simulink model "simulink_flightgear_control_trim_wind_5"  (R2023a)
settings: Solver=VariableStepAuto  StartTime=0  StopTime=inf  FixedStep=0.1  RelTol=1e-3
values from neighbouring files (symbols this model uses):
  model = 'simulink_flightgear_control_trim_wind_5'    [traimcode.m]
  ms2kts = 1.943844492609    (= 1.94384449261)    [Boeing747model.m]    (also in engine.m)
undefined symbols (not defined in the file or in its folder): Earth, F, Light, m, MIL, Model, Newton, Raphson, Receive, s, Send, Unit, WGS84, Wind
libraries: simulink_extras x7, aerolibconvert2 x5, simulink x4, aerolibfltsims x3, shared6dof x1, aerolibasang x1, aerolibtransform2 x1, aerolibatmos2 x1, aerolibobsolete x1, aerolibwind2 x1
(part 2 of 2)

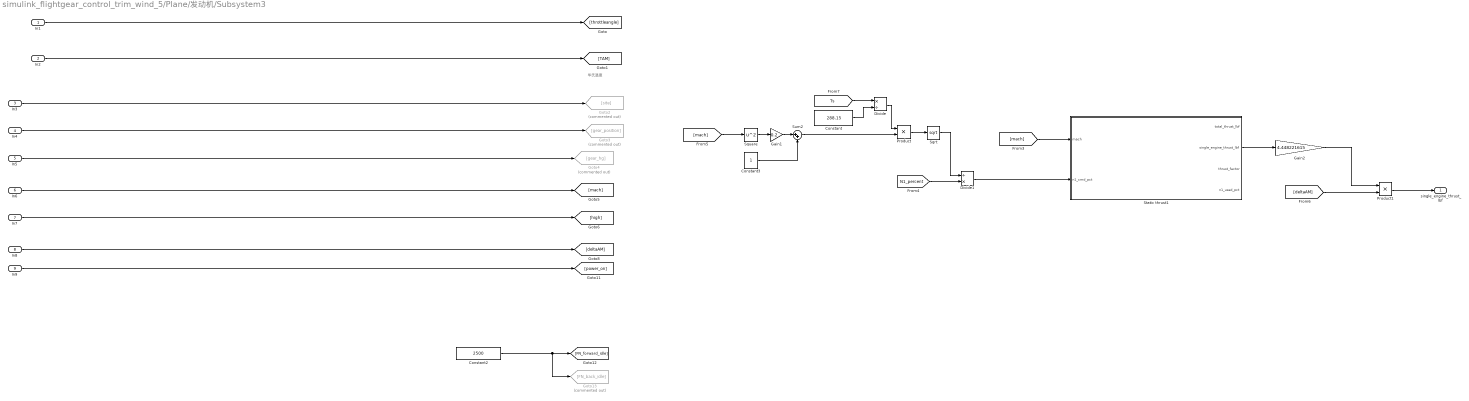
== system simulink_flightgear_control_trim_wind_5/Plane/发动机/Subsystem3 ==
  note: 华氏温度
  In1 : Inport
  In2 : Inport  Port=2
  In3 : Inport  Port=3
  In4 : Inport  Port=4
  In5 : Inport  Port=5
  In6 : Inport  Port=6
  In7 : Inport  Port=7
  In8 : Inport  Port=8
  In9 : Inport  Port=9
  Constant : Constant  Value=288.15
  Constant2 : Constant  Value=2500
  Constant3 : Constant
  Divide : Product  Inputs=*/
  Divide1 : Product  Inputs=/*
  Gain1 : Gain  Gain=0.2
  Gain2 : Gain  Gain=4.448221615
  Goto13 : Goto  Commented=on  GotoTag=FN_back_idle
  Goto2 : Goto  Commented=on  GotoTag=site
  Goto3 : Goto  Commented=on  GotoTag=gear_position
  Goto4 : Goto  Commented=on  GotoTag=gear_hg
  Product : Product
  Product1 : Product
  Sqrt : Sqrt
  Square : Math  Operator=square
  Static thrust1 : MATLAB Function  TreatAsAtomicUnit=on
  Sum2 : Sum  Inputs=|++
  single_engine_thrust_lbf : Outport
  wires:
  In2/1 -> [TAM]
  In1/1 -> [throttleangle]
  In5/1 -> Goto4/1
  In3/1 -> Goto2/1
  In4/1 -> Goto3/1
  In6/1 -> [mach]
  In8/1 -> [deltaAM]
  In7/1 -> [high]
  In9/1 -> [power_on]
  Constant2/1 -> [FN_forward_idle], Goto13/1
  Product1/1 -> single_engine_thrust_lbf/1
  [N1_percent] -> Divide1/2
  Divide1/1 -> Static thrust1/2(n1_cmd_pct)
  Divide/1 -> Product/1
  [mach] -> Square/1
  [Ts] -> Divide/1
  Constant3/1 -> Sum2/2
  [mach] -> Static thrust1/1(mach)
  Constant/1 -> Divide/2
  Gain1/1 -> Sum2/1
  Sum2/1 -> Product/2
  Square/1 -> Gain1/1
  Sqrt/1 -> Divide1/1
  Product/1 -> Sqrt/1
  [deltaAM] -> Product1/2
  Static thrust1/2(single_engine_thrust_lbf) -> Gain2/1
  Gain2/1 -> Product1/1

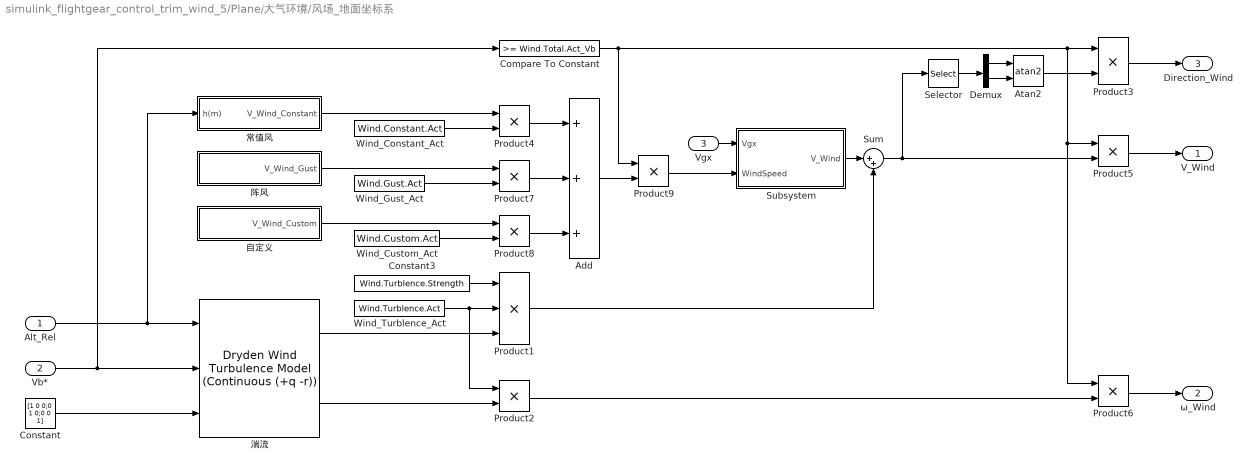
== system simulink_flightgear_control_trim_wind_5/Plane/大气环境/风场_地面坐标系 ==
  Alt_Rel : Inport
  Vb* : Inport  Port=2
  Vgx : Inport  Port=3
  Add : Sum  Inputs=+++
  Atan2 : Trigonometry  Operator=atan2
  Compare To Constant : simulink/Logic and Bit Operations/Compare To Constant  relop=>=  const=Wind.Total.Act_Vb  OutDataTypeStr=uint8
  Constant : Constant  Value=[1 0 0;0 1 0;0 0 1]
  Constant3 : Constant  Value=Wind.Turblence.Strength
  Demux : Demux  Outputs=2
  Product1 : Product  Inputs=3
  Product{2..9} (8 alike) : Product
  Selector : Selector  InputPortWidth=3  IndexOptions=Index vector (dialog)  Indices=[2 1]  OutputSizes=1
  Subsystem : Subsystem
  Sum : Sum  Inputs=|++
  Wind_Constant_Act : Constant  Value=Wind.Constant.Act
  Wind_Custom_Act : Constant  Value=Wind.Custom.Act
  Wind_Gust_Act : Constant  Value=Wind.Gust.Act
  Wind_Turblence_Act : Constant  Value=Wind.Turblence.Act
  常值风 : Subsystem
  湍流 : aerolibwind2/Dryden Wind Turbulence Model  (Continuous (+q -r))  units=Metric (MKS)  spec=MIL-F-8785C  model=Continuous Dryden (+q +r)  W20=Wind.Constant.Vxy_Ground  Wdeg=Wind.Constant.Direction  TurbProb=10^-2 - Light  L_high=533.4  Wingspan=Model.b  ts=Wind.Turblence.SampleTime  Seed=[fix(rand(1,1)*25000), fix(rand(1,1)*25000+1), fix(rand(1,1)*25000+2), fix(rand(1,1)*25000+3)]  T_on=on
  自定义 : Subsystem
  阵风 : Subsystem
  V_Wind : Outport  VectorParamsAs1DForOutWhenUnconnected=off
  ω_Wind : Outport  Port=2  VectorParamsAs1DForOutWhenUnconnected=off
  Direction_Wind : Outport  Port=3  VectorParamsAs1DForOutWhenUnconnected=off
  wires:
  Wind_Custom_Act/1 -> Product8/2
  Product8/1 -> Add/3
  自定义/1(V_Wind_Custom) -> Product8/1
  Wind_Turblence_Act/1 -> Product2/1, Product1/2
  Wind_Gust_Act/1 -> Product7/2
  Wind_Constant_Act/1 -> Product4/2
  Demux/1 -> Atan2/1
  Demux/2 -> Atan2/2
  Selector/1 -> Demux/1
  Compare To Constant/1 -> Product9/1, Product6/1, Product5/1, Product3/1
  Atan2/1 -> Product3/2
  Subsystem/1(V_Wind) -> Sum/1
  Sum/1 -> Product5/2, Selector/1
  Product7/1 -> Add/2
  阵风/1(V_Wind_Gust) -> Product7/1
  Product4/1 -> Add/1
  Product1/1 -> Sum/2
  Product3/1 -> Direction_Wind/1
  Product2/1 -> Product6/2
  Constant3/1 -> Product1/1
  Product6/1 -> ω_Wind/1
  Product5/1 -> V_Wind/1
  Constant/1 -> 湍流/3
  常值风/1(V_Wind_Constant) -> Product4/1
  Vb*/1 -> Compare To Constant/1, 湍流/2
  湍流/2 -> Product2/2
  湍流/1 -> Product1/3
  Alt_Rel/1 -> 常值风/1(h(m)), 湍流/1
  Vgx/1 -> Subsystem/1(Vgx)
  Product9/1 -> Subsystem/2(WindSpeed)
  Add/1 -> Product9/2

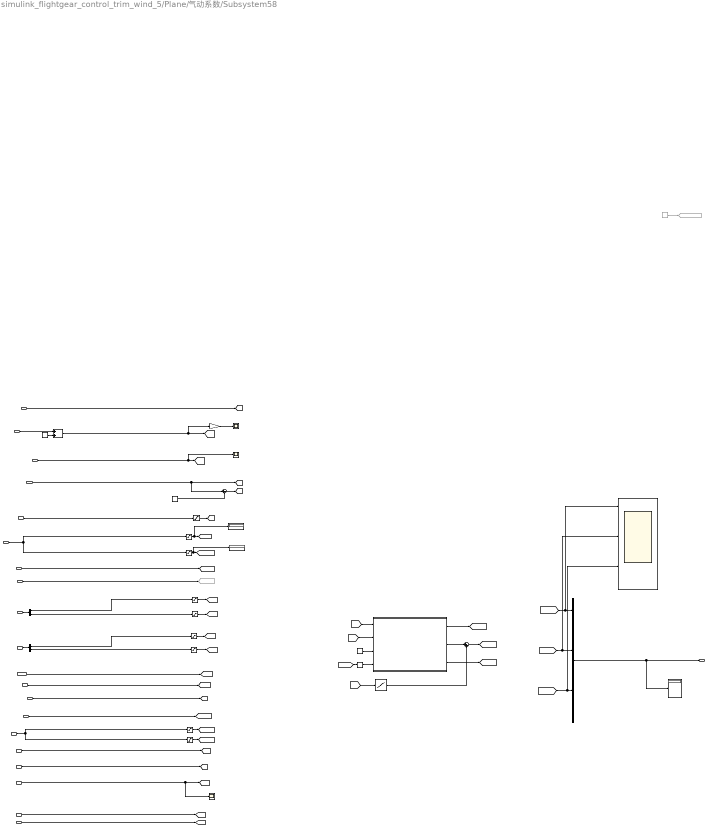
== system simulink_flightgear_control_trim_wind_5/Plane/气动系数/Subsystem58 ==
  note: degree
  note: 输入单位:
      | 角度：弧度
      | 角速度：rad/s
      | 速度:mach
      | 舵面：rad
      | 襟翼：0-1
      | 高度：米
      | 重心：百分比
  note: 内侧升降舵偏转角度
  note: 平尾配平角度
  note: 迎角RAD+安装角
      | 安装角
  note: 外侧升降舵偏转角度
  note: 起落架时间控制系统
  In1 : Inport
  In2 : Inport  Port=2
  In3 : Inport  Port=3
  In4 : Inport  Port=4
  In5 : Inport  Port=5
  In6 : Inport  Port=6
  trim : Inport  Port=7
  In8 : Inport  Port=8
  aere_o : Inport  Port=9
  In10 : Inport  Port=10
  In11 : Inport  Port=11
  In12 : Inport  Port=12
  In13 : Inport  Port=13
  In14 : Inport  Port=14
  In15 : Inport  Port=15
  In16 : Inport  Port=16
  In17 : Inport  Port=17
  In18 : Inport  Port=18
  V_E : Inport  Port=19
  In20 : Inport  Port=20
  2-D Lookup Table : Lookup_n-D  NumberOfTableDimensions=1  BreakpointsForDimension1="[0.0 0.2 0.3 0.4 0.5 0.6 0.7  0.8 0.9 1 1.1 1.2 1.3 3]"  BreakpointsForDimension2=[1:3]  Table="[0   0   0   0   0   0   0.002 0.008 0.02 0.045 0.08 0.045 0.03 0.03]"  InternalRulePriority=Speed  RndMeth=Simplest
  Bus Creator : BusCreator  Inputs=6
  Constant : Constant  Value=0.03490658504
  Constant11 : Constant  Value=0
  Constant4 : Constant  Value=4.58
  Constant5 : Constant  Commented=on  Value=0
  Degrees to Radians : simulink_extras/Transformations/Degrees to Radians
  Demux : Demux  Outputs=2
  Demux1 : Demux  Outputs=2
  Display : Display
  Display1 : Display
  Display2 : Display
  Gain1 : Gain  Gain=57.3
  Goto19 : Goto  Commented=on  GotoTag=gear_position
  Goto35 : Goto  Commented=on  GotoTag=K
  Saturation1 : Saturate  UpperLimit=0.26  LowerLimit=-0.436
  Saturation10 : Saturate  UpperLimit=0.26  LowerLimit=-0.436
  Saturation12 : Saturate  UpperLimit=33  LowerLimit=14
  Saturation14 : Saturate  UpperLimit=0.436  LowerLimit=-0.436
  Saturation16 : Saturate  UpperLimit=0.436  LowerLimit=-0.436
  Saturation3 : Saturate  UpperLimit=0.349  LowerLimit=-0.349
  Saturation4 : Saturate  UpperLimit=0.349  LowerLimit=-0.349
  Saturation8 : Saturate  UpperLimit=0.4  LowerLimit=-0.296
  Saturation9 : Saturate  UpperLimit=0.4  LowerLimit=-0.296
  Scope10 : Scope  NumInputPorts=6
  Scope11 : Scope
  Scope12 : Scope
  Scope16 : Scope
  Static longitudinal aero : MATLAB Function  TreatAsAtomicUnit=on
  Sum : Sum  Inputs=|++
  Sum13 : Sum  Inputs=|+-
  Sum5 : Sum
  Coefficients1 : Outport
  tag scope: V=global
  wires:
  In2/1 -> Sum5/1  "alpha"
  In17/1 -> [r]  "r"
  In6/1 -> Saturation8/1, Saturation9/1  "Elevators"
  In10/1 -> [dot_alpha]  "dot_alpha"
  Saturation12/1 -> [cg]
  In13/1 -> [beta]  "beta"
  Saturation8/1 -> Display1/1, [delta_ei]
  In5/1 -> Saturation12/1  "cg"
  In8/1 -> Goto19/1  "gear_position"
  In1/1 -> [flap]  "flap"
  In11/1 -> [q]  "q"
  In16/1 -> [p]  "p"
  In3/1 -> Scope12/1, [mach]  "mach"
  Saturation16/1 -> [rudder_l]
  Saturation14/1 -> [rudder_u]
  In4/1 -> [high], Sum13/1  "high"
  trim/1 -> [delta_FRL]
  In14/1 -> Saturation14/1, Saturation16/1  "rudder"
  Saturation9/1 -> Display2/1, [delta_eo]
  In18/1 -> Scope16/1, [dot_beta]  "dot_beta"
  In12/1 -> [nz]  "nz"
  Constant/1 -> Sum5/2
  Sum5/1 -> Gain1/1, [alpha]
  V_E/1 -> [V_E]
  In20/1 -> [V]  "V"
  [CM] -> Scope10/5, Bus Creator/5
  [CL] -> Scope10/3, Bus Creator/3
  Bus Creator/1 -> Display/1, Coefficients1/1  "parameter"
  [CD] -> Scope10/1, Bus Creator/1
  Gain1/1 -> Scope11/1
  Demux/1 -> Saturation10/1
  Demux/2 -> Saturation1/1
  In15/1 -> Demux1/1  "ai"
  Saturation3/1 -> [aerol_in_l]
  Demux1/2 -> Saturation4/1
  Saturation4/1 -> [aerol_in_r]
  Saturation10/1 -> [left_aero]
  Demux1/1 -> Saturation3/1
  aere_o/1 -> Demux/1
  Saturation1/1 -> [right_aero]
  Sum13/1 -> [high_g]
  Constant4/1 -> Sum13/2
  Constant5/1 -> Goto35/1
  [alpha] -> Static longitudinal aero/1(alpha_rad)
  Static longitudinal aero/1(CL) -> [CL]
  Constant11/1 -> Static longitudinal aero/3(elevator_rad)
  [mach] -> Static longitudinal aero/2(mach)
  [delta_FRL] -> Degrees to Radians/1
  Degrees to Radians/1 -> Static longitudinal aero/4(elevator_trim_rad)
  Static longitudinal aero/3(CM) -> [CM]
  Static longitudinal aero/2(CD) -> Sum/1
  Sum/1 -> [CD]
  [mach] -> 2-D Lookup Table/1
  2-D Lookup Table/1 -> Sum/2

== system simulink_flightgear_control_trim_wind_5/Plane/参数计算/Subsystem1/Subsystem ==
  Vb : Inport
  Demux1 : Demux  Outputs=3
      settings: DisplayOption=none
  Terminator : Terminator
  w : Outport  VectorParamsAs1DForOutWhenUnconnected=off
  u : Outport  Port=2  VectorParamsAs1DForOutWhenUnconnected=off
  wires:
  Demux1/2 -> Terminator/1
  Vb/1 -> Demux1/1
  Demux1/1 -> u/1
  Demux1/3 -> w/1

== system simulink_flightgear_control_trim_wind_5/Plane/参数计算/Subsystem1/Subsystem1 ==
  Vb : Inport
  Demux1 : Demux  Outputs=3
      settings: DisplayOption=none
  Terminator : Terminator
  Terminator1 : Terminator
  v : Outport  VectorParamsAs1DForOutWhenUnconnected=off
  wires:
  Demux1/3 -> Terminator1/1
  Demux1/1 -> Terminator/1
  Demux1/2 -> v/1
  Vb/1 -> Demux1/1

== system simulink_flightgear_control_trim_wind_5/Plane/参数计算/Subsystem1/Subsystem2 ==
  Vb : Inport
  Demux1 : Demux  Outputs=3
  Product1 : Product  RndMeth=Zero
  Product2 : Product  RndMeth=Zero
  Product3 : Product  RndMeth=Zero
  Sum : Sum  Inputs=+++
  u²+v²+w² : Outport  VectorParamsAs1DForOutWhenUnconnected=off
  wires:
  Demux1/1 -> Product1/1, Product1/2
  Product1/1 -> Sum/1
  Sum/1 -> u²+v²+w²/1
  Demux1/3 -> Product3/1, Product3/2
  Vb/1 -> Demux1/1
  Product2/1 -> Sum/2
  Demux1/2 -> Product2/2, Product2/1
  Product3/1 -> Sum/3

== system simulink_flightgear_control_trim_wind_5/Plane/参数计算/航迹角/Subsystem ==
  Vg : Inport
  Demux1 : Demux  Outputs=3
      settings: DisplayOption=none
  Terminator : Terminator
  Vy : Outport  VectorParamsAs1DForOutWhenUnconnected=off
  Vx : Outport  Port=2  VectorParamsAs1DForOutWhenUnconnected=off
  wires:
  Vg/1 -> Demux1/1
  Demux1/1 -> Vx/1
  Demux1/3 -> Terminator/1
  Demux1/2 -> Vy/1

== system simulink_flightgear_control_trim_wind_5/Plane/参数计算/航迹角/Subsystem1 ==
  Vg : Inport
  Demux1 : Demux  Outputs=3
      settings: DisplayOption=none
  Terminator : Terminator
  Terminator1 : Terminator
  Vz : Outport  VectorParamsAs1DForOutWhenUnconnected=off
  wires:
  Demux1/1 -> Terminator/1
  Vg/1 -> Demux1/1
  Demux1/3 -> Vz/1
  Demux1/2 -> Terminator1/1

== system simulink_flightgear_control_trim_wind_5/Plane/参数计算/航迹角/Subsystem3 ==
  Vg : Inport
  Demux2 : Demux  Outputs=3
  Product : Product  RndMeth=Zero
  Product1 : Product  RndMeth=Zero
  Sum : Sum  Inputs=++|
  Terminator1 : Terminator
  Vx²+Vy² : Outport  VectorParamsAs1DForOutWhenUnconnected=off
  wires:
  Product1/1 -> Sum/2
  Demux2/1 -> Product/1, Product/2
  Vg/1 -> Demux2/1
  Demux2/2 -> Product1/1, Product1/2
  Product/1 -> Sum/1
  Sum/1 -> Vx²+Vy²/1
  Demux2/3 -> Terminator1/1

== system simulink_flightgear_control_trim_wind_5/Plane/大气环境/风场_地面坐标系/Subsystem ==
  Vgx : Inport
  WindSpeed : Inport  Port=2
  Abs : Abs  SaturateOnIntegerOverflow=off
  Constant2 : Constant  Value=Wind.Total.Length
  Divide : Product  Inputs=*/
  Rate Limiter Dynamic : simulink/Discontinuities/Rate Limiter Dynamic
  Saturation : Saturate  UpperLimit=inf  LowerLimit=Wind.Total.GrowRate_Min
  Saturation1 : Saturate  UpperLimit=-Wind.Total.GrowRate_Min  LowerLimit=-inf
  Unary Minus : UnaryMinus
  V_Wind : Outport  VectorParamsAs1DForOutWhenUnconnected=off
  wires:
  Saturation1/1 -> Rate Limiter Dynamic/3
  Saturation/1 -> Rate Limiter Dynamic/1
  Abs/1 -> Divide/1
  Unary Minus/1 -> Saturation1/1
  Vgx/1 -> Abs/1
  Divide/1 -> Saturation/1, Unary Minus/1
  Constant2/1 -> Divide/2
  WindSpeed/1 -> Rate Limiter Dynamic/2
  Rate Limiter Dynamic/1 -> V_Wind/1

== system simulink_flightgear_control_trim_wind_5/Plane/大气环境/风场_地面坐标系/常值风 ==
  h(m) : Inport
  Constant : Constant  Value=0
  Fcn : Fcn  Expr=Wind.Constant.Vxy_Ground + (Wind.Constant.Vxy_RefAlt / Wind.Constant.RefAlt^2)
  Gain : Gain  Gain=cos(deg2rad(Wind.Constant.Direction))
  Gain1 : Gain  Gain=sin(deg2rad(Wind.Constant.Direction))
  Mux : Mux  Inputs=3
  V_Wind_Constant : Outport  VectorParamsAs1DForOutWhenUnconnected=off
  wires:
  Mux/1 -> V_Wind_Constant/1
  Gain1/1 -> Mux/2
  Constant/1 -> Mux/3
  Fcn/1 -> Gain/1, Gain1/1
  Gain/1 -> Mux/1
  h(m)/1 -> Fcn/1

== system simulink_flightgear_control_trim_wind_5/Plane/大气环境/风场_地面坐标系/自定义 ==
  Angle Conversion2 : aerolibconvert2/Angle Conversion  IU=deg  OU=rad
  Mux : Mux  Inputs=3
  Product : Product
  Product1 : Product
  Trigonometric Function : Trigonometry  Operator=cos
  Trigonometric Function1 : Trigonometry
  Wind_Custom_Direction : Constant  Value=Wind.Custom.Direction
  Wind_Custom_Vxy : Constant  Value=Wind.Custom.Vxy
  Wind_Custom_Vz : Constant  Value=Wind.Custom.Vz
  V_Wind_Custom : Outport  VectorParamsAs1DForOutWhenUnconnected=off
  wires:
  Angle Conversion2/1 -> Trigonometric Function/1, Trigonometric Function1/1
  Wind_Custom_Vxy/1 -> Product/1, Product1/1
  Trigonometric Function/1 -> Product/2
  Trigonometric Function1/1 -> Product1/2
  Wind_Custom_Direction/1 -> Angle Conversion2/1
  Product/1 -> Mux/1
  Wind_Custom_Vz/1 -> Mux/3
  Product1/1 -> Mux/2
  Mux/1 -> V_Wind_Custom/1

== system simulink_flightgear_control_trim_wind_5/Plane/大气环境/风场_地面坐标系/阵风 ==
  Angle Conversion1 : aerolibconvert2/Angle Conversion  IU=deg  OU=rad
  Constant1 : Constant  Value=Wind.Gust.Vxy_max
  Constant2 : Constant  Value=Wind.Gust.Vz_max
  Constant3 : Constant  Value=Wind.Gust.Act_Random_V
  Constant4 : Constant  Value=Wind.Gust.Direction
  Constant6 : Constant  Value=Wind.Gust.Act_Random_Direction
  Constant7 : Constant  Value=Wind.Gust.Act_Random_V
  Mux : Mux  Inputs=3
  Product : Product
  Product3 : Product
  Product4 : Product
  Pulse Generator : DiscretePulseGenerator  PulseType=Time based  Period=Wind.Gust.SampleTime + Wind.Gust.ContinueTime  PulseWidth=Wind.Gust.ContinueTime / (Wind.Gust.SampleTime + Wind.Gust.ContinueTime) * 100  PhaseDelay=Wind.Gust.SampleTime
  Switch : Switch  Criteria=u2 ~= 0  SaturateOnIntegerOverflow=off  InputSameDT=off
  Switch1 : Switch  Criteria=u2 ~= 0  SaturateOnIntegerOverflow=off  InputSameDT=off
  Switch2 : Switch  Criteria=u2 ~= 0  SaturateOnIntegerOverflow=off  InputSameDT=off
  Trigonometric Function : Trigonometry  Operator=cos
  Trigonometric Function1 : Trigonometry
  Uniform Random Number : UniformRandomNumber  Minimum=Wind.Gust.Vxy_min  Maximum=Wind.Gust.Vxy_max + eps  Seed=fix(rand(1,1)*25000)  SampleTime=Wind.Gust.SampleTime + Wind.Gust.ContinueTime
  Uniform Random Number1 : UniformRandomNumber  Minimum=0  Maximum=360  Seed=fix(rand(1,1)*25000)  SampleTime=Wind.Gust.SampleTime + Wind.Gust.ContinueTime
  Uniform Random Number2 : UniformRandomNumber  Minimum=Wind.Gust.Vz_min  Maximum=Wind.Gust.Vz_max + eps  Seed=fix(rand(1,1)*25000)  SampleTime=Wind.Gust.SampleTime + Wind.Gust.ContinueTime
  V_Wind_Gust : Outport  VectorParamsAs1DForOutWhenUnconnected=off
  wires:
  Uniform Random Number2/1 -> Switch2/1
  Constant7/1 -> Switch2/2
  Angle Conversion1/1 -> Trigonometric Function/1, Trigonometric Function1/1
  Constant4/1 -> Switch1/3
  Uniform Random Number1/1 -> Switch1/1
  Constant6/1 -> Switch1/2
  Trigonometric Function1/1 -> Product4/2
  Trigonometric Function/1 -> Product/2
  Switch/1 -> Product/1, Product4/1
  Switch1/1 -> Angle Conversion1/1
  Mux/1 -> Product3/1
  Constant2/1 -> Switch2/3
  Constant3/1 -> Switch/2
  Switch2/1 -> Mux/3
  Uniform Random Number/1 -> Switch/1
  Constant1/1 -> Switch/3
  Pulse Generator/1 -> Product3/2
  Product4/1 -> Mux/2
  Product/1 -> Mux/1
  Product3/1 -> V_Wind_Gust/1

== matlab function simulink_flightgear_control_trim_wind_5/Plane/气动力//力矩/MATLAB Function ==
  data: u input; y output
function y = fcn(u)

x = [cosd(u) 0 -sind(u); %x为稳定轴系到体轴系的转换
    0       1      0 ;
    sind(u) 0  cosd(u)];

y=x;

== matlab function simulink_flightgear_control_trim_wind_5/Plane/发动机/MATLAB Function4 ==
  data: u input; y output
function y = fcn(u)

y = u*9/5-459.67;

== matlab function simulink_flightgear_control_trim_wind_5/Plane/发动机/MATLAB Function ==
  data: x input; T output; y input; z input
function T = fcn(x,y,z)

T= [x,y,z]';

== matlab function simulink_flightgear_control_trim_wind_5/Plane/发动机/MATLAB Function1 ==
  data: x input; MT output; y input; z input
function MT = fcn(x,y,z)

MT= [x,y,z]';

== matlab function simulink_flightgear_control_trim_wind_5/Plane/发动机/MATLAB Function2 ==
  data: flap input; site output; ma input
function site= fcn(flap,ma)
if(ma>=0&&ma<=0.25)
    if(flap==0)
    site=0;
    elseif (flap>0.1&&flap<=0.25)
        site=1;
    elseif(flap>0.25&&flap<=0.5)
        site=2;
    elseif(flap>0.5&&flap<=0.75)
        site=3;
    elseif(flap>0.75&&flap<=1)
        site=4;
    else
    site=0;
    end
elseif(ma>0.25&&ma<=0.35)
    if(flap==0)
    site=0;
    elseif(flap>0.1&&flap<=0.25)
        site=1;
    elseif(flap>0.25&&flap<=0.5)
        site=2;
    elseif(flap>0.5)
        site=3;
    else
    site=0;
    end
else
    site=0;
end

== matlab function simulink_flightgear_control_trim_wind_5/Plane/重量//惯量/MATLAB Function1 ==
  data: ixx input; y output; iyy input; izz input; ixz input
function y = fcn(ixx,iyy,izz,ixz)
I=[ixx  0  -ixz;
    0  iyy  0;
    -ixz 0   izz];
y = I;

== matlab function simulink_flightgear_control_trim_wind_5/Plane/MATLAB Function ==
  data: u input; y output
function y = fcn(u)

y = [(25-u)/100*8.32,0,0]';

== matlab function simulink_flightgear_control_trim_wind_5/Plane/气动系数/MATLAB Function ==
  data: u input; y output
function y = fcn(u)

x = [cosd(u) 0 -sind(u); %x为稳定轴系到体轴系的转换
    0       1      0 ;
    sind(u) 0  cosd(u)];

y=x';                  %y为体轴系到稳定轴系的转换

== matlab function simulink_flightgear_control_trim_wind_5/Plane/大气环境/气压高度+摄氏度偏差版本1 ==
  data: T output; p output; rho output; Hp input; a output; delta_ISA input; delta output; theta output; sigma output; Hd_m output; Hd_ft output
% File: isa_atmosphere_pressure_altitude_delta.m
%
% 输入:
%   Hp        气压高度 / pressure altitude (m) [0–84.852 km]
%   delta_ISA 温度偏差 (degC)，比如 -40 表示 ISA -40
%
% 输出:
%   T     实际温度 (K)，即 T_ISA(Hp) + delta_ISA
%   p     静压 (Pa)，由气压高度按 ISA 标准大气确定
%   rho   实际密度 (kg/m^3)，由 p 和 T 计算
%   a     实际声速 (m/s)，由 T 计算
%   delta 压力比 p/p0
%   theta 温度比 T/T0
%   sigma 密度比 rho/rho0
%   Hd_m  密度高度 (m)
%   Hd_ft 密度高度 (ft)

function [T, p, rho, a, delta, theta, sigma, Hd_m, Hd_ft] = isa_atmosphere_pressure_altitude_delta(Hp, delta_ISA)

    % 常数
    g0 = 9.80665;        % m/s^2
    R  = 287.05287;      % J/(kg*K)
    gamma = 1.4;         % 空气比热比

    p0 = 101325;         % Pa
    T0 = 288.15;         % K
    rho0 = 1.225;        % kg/m^3

    % ISA 分层参数
    h_base = [0, 11000, 20000, 32000, 47000, 51000, 71000, 84852]; % m
    L      = [-0.0065, 0.0, 0.0010, 0.0028, 0.0, -0.0028, -0.0020]; % K/m

    % 输入检查
    if any(Hp(:) < 0) || any(Hp(:) > 84852)
        error('Hp must be within [0, 84852] m.');
    end

    if isscalar(delta_ISA)
        delta_ISA = delta_ISA .* ones(size(Hp));
    elseif ~isequal(size(delta_ISA), size(Hp))
        error('delta_ISA must be scalar or the same size as Hp.');
    end

    T_ISA = zeros(size(Hp));
    p     = zeros(size(Hp));

    % 对每一个气压高度计算 ISA 温度和 ISA 压力
    for i = 1:numel(Hp)

        h = Hp(i);

        T_curr = T0;
        p_curr = p0;

        for j = 1:length(L)

            h1 = h_base(j);
            h2 = h_base(j+1);

            if h <= h2

                if L(j) == 0
                    T_layer = T_curr;
                    p(i) = p_curr * exp(-g0 * (h - h1) / (R * T_layer));
                else
                    T_layer = T_curr + L(j) * (h - h1);
                    p(i) = p_curr * (T_layer / T_curr)^(-g0 / (R * L(j)));
                end

                T_ISA(i) = T_layer;
                break;

            else

                if L(j) == 0
                    T_next = T_curr;
                    p_curr = p_curr * exp(-g0 * (h2 - h1) / (R * T_curr));
                else
                    T_next = T_curr + L(j) * (h2 - h1);
                    p_curr = p_curr * (T_next / T_curr)^(-g0 / (R * L(j)));
                end

                T_curr = T_next;
            end
        end
    end

    % 实际温度：ISA 温度 + ΔISA
    T = T_ISA + delta_ISA;

    if any(T(:) <= 0)
        error('Computed temperature is non-physical. T must be greater than 0 K.');
    end

    % 实际密度和声速
    rho = p ./ (R .* T);
    a   = sqrt(gamma * R .* T);

    % 无量纲比值
    delta = p ./ p0;
    theta = T ./ T0;
    sigma = rho ./ rho0;

    % 密度高度
    Hd_m = density_altitude_from_rho(rho);
    Hd_ft = Hd_m * 3.280839895;
end


function Hd = density_altitude_from_rho(rho_target)

    h_low  = -3048;   % -10000 ft
    h_high = 15240;   %  50000 ft

    Hd = zeros(size(rho_target));

    for i = 1:numel(rho_target)
        lo = h_low;
        hi = h_high;

        for k = 1:60
            mid = 0.5 * (lo + hi);
            rho_mid = isa_density(mid);

            if rho_mid > rho_target(i)
                lo = mid;
            else
                hi = mid;
            end
        end

        Hd(i) = 0.5 * (lo + hi);
    end
end


function rho = isa_density(h)
    [T, p] = isa_standard_Tp(h);
    R = 287.05287;
    rho = p / (R * T);
end


function [T, p] = isa_standard_Tp(h)

    g0 = 9.80665;
    R  = 287.05287;

    p0 = 101325;
    T0 = 288.15;

    h_base = [0, 11000, 20000, 32000, 47000, 51000, 71000, 84852];
    L      = [-0.0065, 0.0, 0.0010, 0.0028, 0.0, -0.0028, -0.0020];

    % 默认赋值，避免 Simulink Coder 认为输出未赋值
    T = T0;
    p = p0;

    T_curr = T0;
    p_curr = p0;

    for j = 1:length(L)
        h1 = h_base(j);
        h2 = h_base(j+1);

        if h <= h2
            if L(j) == 0
                T = T_curr;
                p = p_curr * exp(-g0 * (h - h1) / (R * T));
            else
                T = T_curr + L(j) * (h - h1);
                p = p_curr * (T / T_curr)^(-g0 / (R * L(j)));
            end
            return;
        else
            if L(j) == 0
                T_next = T_curr;
                p_curr = p_curr * exp(-g0 * (h2 - h1) / (R * T_curr));
            else
                T_next = T_curr + L(j) * (h2 - h1);
                p_curr = p_curr * (T_next / T_curr)^(-g0 / (R * L(j)));
            end

            T_curr = T_next;
        end
    end

    % 兜底路径，给 Coder 明确输出
    T = T_curr;
    p = p_curr;
end

== matlab function simulink_flightgear_control_trim_wind_5/Plane/发动机/Subsystem1/Static thrust1 ==
  data: mach input; total_thrust_lbf output; n1_cmd_pct input; single_engine_thrust_lbf output; thrust_factor output; n1_used_pct output
function [total_thrust_lbf, single_engine_thrust_lbf, thrust_factor, n1_used_pct] = core(mach, n1_cmd_pct)
%#codegen
n1_bp = [0 20 25 30 35 40 45 50 55 60 65 70 75 80 85 90 95 100 105 110];
mach_bp = [0 0.45 0.9];
tf_tbl = [0 0 0;0.053978 0.034816 0.080724;0.072647 0.042137 0.153968;0.092571 0.055766 0.352444;0.114397 0.087857 0.382598;0.133584 0.129235 0.401433;0.163657 0.179995 0.424077;0.201611 0.227881 0.453427;0.247145 0.284959 0.489514;0.306598 0.357671 0.526682;0.404374 0.458374 0.565243;0.472288 0.53715 0.610145;0.543975 0.608862 0.67375;0.628349 0.697486 0.766623;0.735036 0.796225 0.857414;0.837808 0.906299 0.97479;0.956614 1.020258 1.083902;1.090953 1.156054 1.221156;1.234866 1.296368 1.35787;1.325555 1.380287 1.43502];
static_thrust = 66500;
thrust_scalar = 1;
thrust_limit = 1;
n1_used_pct = min(max(n1_cmd_pct, n1_bp(1)), n1_bp(end));
thrust_factor = lookup2(n1_bp, mach_bp, tf_tbl, n1_used_pct, mach);
single_engine_thrust_lbf = static_thrust * thrust_factor * thrust_scalar * thrust_limit;
total_thrust_lbf = 4.0 * single_engine_thrust_lbf;
end

function v = lookup1(xbp, ybp, x)
x = min(max(x, xbp(1)), xbp(end));
idx = findInterval(xbp, x);
x1 = xbp(idx); x2 = xbp(idx+1);
t = 0.0;
if x2 ~= x1
    t = (x - x1) / (x2 - x1);
end
v = ybp(idx) + t * (ybp(idx+1) - ybp(idx));
end

function v = lookup2(xbp, ybp, table, x, y)
x = min(max(x, xbp(1)), xbp(end));
y = min(max(y, ybp(1)), ybp(end));
ix = findInterval(xbp, x);
iy = findInterval(ybp, y);
x1 = xbp(ix); x2 = xbp(ix+1);
y1 = ybp(iy); y2 = ybp(iy+1);
tx = 0.0; ty = 0.0;
if x2 ~= x1
    tx = (x - x1) / (x2 - x1);
end
if y2 ~= y1
    ty = (y - y1) / (y2 - y1);
end
q11 = table(ix, iy);
q21 = table(ix+1, iy);
q12 = table(ix, iy+1);
q22 = table(ix+1, iy+1);
v = (1-tx)*(1-ty)*q11 + tx*(1-ty)*q21 + (1-tx)*ty*q12 + tx*ty*q22;
end

function idx = findInterval(bp, x)
idx = 1;
for n = 1:(numel(bp)-1)
    if x >= bp(n) && x <= bp(n+1)
        idx = n;
        return;
    end
end
idx = numel(bp)-1;
end

== matlab function simulink_flightgear_control_trim_wind_5/Plane/发动机/Subsystem2/Static thrust1 ==
  data: mach input; total_thrust_lbf output; n1_cmd_pct input; single_engine_thrust_lbf output; thrust_factor output; n1_used_pct output
function [total_thrust_lbf, single_engine_thrust_lbf, thrust_factor, n1_used_pct] = core(mach, n1_cmd_pct)
%#codegen
n1_bp = [0 20 25 30 35 40 45 50 55 60 65 70 75 80 85 90 95 100 105 110];
mach_bp = [0 0.45 0.9];
tf_tbl = [0 0 0;0.053978 0.034816 0.080724;0.072647 0.042137 0.153968;0.092571 0.055766 0.352444;0.114397 0.087857 0.382598;0.133584 0.129235 0.401433;0.163657 0.179995 0.424077;0.201611 0.227881 0.453427;0.247145 0.284959 0.489514;0.306598 0.357671 0.526682;0.404374 0.458374 0.565243;0.472288 0.53715 0.610145;0.543975 0.608862 0.67375;0.628349 0.697486 0.766623;0.735036 0.796225 0.857414;0.837808 0.906299 0.97479;0.956614 1.020258 1.083902;1.090953 1.156054 1.221156;1.234866 1.296368 1.35787;1.325555 1.380287 1.43502];
static_thrust = 66500;
thrust_scalar = 1;
thrust_limit = 1;
n1_used_pct = min(max(n1_cmd_pct, n1_bp(1)), n1_bp(end));
thrust_factor = lookup2(n1_bp, mach_bp, tf_tbl, n1_used_pct, mach);
single_engine_thrust_lbf = static_thrust * thrust_factor * thrust_scalar * thrust_limit;
total_thrust_lbf = 4.0 * single_engine_thrust_lbf;
end

function v = lookup1(xbp, ybp, x)
x = min(max(x, xbp(1)), xbp(end));
idx = findInterval(xbp, x);
x1 = xbp(idx); x2 = xbp(idx+1);
t = 0.0;
if x2 ~= x1
    t = (x - x1) / (x2 - x1);
end
v = ybp(idx) + t * (ybp(idx+1) - ybp(idx));
end

function v = lookup2(xbp, ybp, table, x, y)
x = min(max(x, xbp(1)), xbp(end));
y = min(max(y, ybp(1)), ybp(end));
ix = findInterval(xbp, x);
iy = findInterval(ybp, y);
x1 = xbp(ix); x2 = xbp(ix+1);
y1 = ybp(iy); y2 = ybp(iy+1);
tx = 0.0; ty = 0.0;
if x2 ~= x1
    tx = (x - x1) / (x2 - x1);
end
if y2 ~= y1
    ty = (y - y1) / (y2 - y1);
end
q11 = table(ix, iy);
q21 = table(ix+1, iy);
q12 = table(ix, iy+1);
q22 = table(ix+1, iy+1);
v = (1-tx)*(1-ty)*q11 + tx*(1-ty)*q21 + (1-tx)*ty*q12 + tx*ty*q22;
end

function idx = findInterval(bp, x)
idx = 1;
for n = 1:(numel(bp)-1)
    if x >= bp(n) && x <= bp(n+1)
        idx = n;
        return;
    end
end
idx = numel(bp)-1;
end

== matlab function simulink_flightgear_control_trim_wind_5/Plane/发动机/Subsystem3/Static thrust1 ==
  data: mach input; total_thrust_lbf output; n1_cmd_pct input; single_engine_thrust_lbf output; thrust_factor output; n1_used_pct output
function [total_thrust_lbf, single_engine_thrust_lbf, thrust_factor, n1_used_pct] = core(mach, n1_cmd_pct)
%#codegen
n1_bp = [0 20 25 30 35 40 45 50 55 60 65 70 75 80 85 90 95 100 105 110];
mach_bp = [0 0.45 0.9];
tf_tbl = [0 0 0;0.053978 0.034816 0.080724;0.072647 0.042137 0.153968;0.092571 0.055766 0.352444;0.114397 0.087857 0.382598;0.133584 0.129235 0.401433;0.163657 0.179995 0.424077;0.201611 0.227881 0.453427;0.247145 0.284959 0.489514;0.306598 0.357671 0.526682;0.404374 0.458374 0.565243;0.472288 0.53715 0.610145;0.543975 0.608862 0.67375;0.628349 0.697486 0.766623;0.735036 0.796225 0.857414;0.837808 0.906299 0.97479;0.956614 1.020258 1.083902;1.090953 1.156054 1.221156;1.234866 1.296368 1.35787;1.325555 1.380287 1.43502];
static_thrust = 66500;
thrust_scalar = 1;
thrust_limit = 1;
n1_used_pct = min(max(n1_cmd_pct, n1_bp(1)), n1_bp(end));
thrust_factor = lookup2(n1_bp, mach_bp, tf_tbl, n1_used_pct, mach);
single_engine_thrust_lbf = static_thrust * thrust_factor * thrust_scalar * thrust_limit;
total_thrust_lbf = 4.0 * single_engine_thrust_lbf;
end

function v = lookup1(xbp, ybp, x)
x = min(max(x, xbp(1)), xbp(end));
idx = findInterval(xbp, x);
x1 = xbp(idx); x2 = xbp(idx+1);
t = 0.0;
if x2 ~= x1
    t = (x - x1) / (x2 - x1);
end
v = ybp(idx) + t * (ybp(idx+1) - ybp(idx));
end

function v = lookup2(xbp, ybp, table, x, y)
x = min(max(x, xbp(1)), xbp(end));
y = min(max(y, ybp(1)), ybp(end));
ix = findInterval(xbp, x);
iy = findInterval(ybp, y);
x1 = xbp(ix); x2 = xbp(ix+1);
y1 = ybp(iy); y2 = ybp(iy+1);
tx = 0.0; ty = 0.0;
if x2 ~= x1
    tx = (x - x1) / (x2 - x1);
end
if y2 ~= y1
    ty = (y - y1) / (y2 - y1);
end
q11 = table(ix, iy);
q21 = table(ix+1, iy);
q12 = table(ix, iy+1);
q22 = table(ix+1, iy+1);
v = (1-tx)*(1-ty)*q11 + tx*(1-ty)*q21 + (1-tx)*ty*q12 + tx*ty*q22;
end

function idx = findInterval(bp, x)
idx = 1;
for n = 1:(numel(bp)-1)
    if x >= bp(n) && x <= bp(n+1)
        idx = n;
        return;
    end
end
idx = numel(bp)-1;
end

== matlab function simulink_flightgear_control_trim_wind_5/Plane/气动系数/Subsystem58/Static longitudinal aero ==
  data: alpha_rad input; CL output; mach input; elevator_rad input; elevator_trim_rad input; CD output; CM output
function [CL, CD, CM] = core(alpha_rad, mach, elevator_rad, elevator_trim_rad)
%#codegen
lift_x = [-3.15 -0.8 -0.4 -0.2 -0.1 0 0.14 0.16 0.176 0.19 3.15]; lift_y = [0 -1.154 -0.928 -0.781 -0.262 0.23 1.009 1.13 1.233 0.35 0];
pitch_x = [-3.15 -0.8 -0.4 -0.2 -0.1 0 0.2 0.23 0.26 0.29 0.31 0.4 0.8 3.15]; pitch_y = [0 -1.767 -0.918 -0.833 -0.555 0 0.964 1.003 1.024 1.116 1.08 1.046 1.745 0];
elev_eff_x = [-180 -40 -20 -14 -7 0 7 14 20 40 180]; elev_eff_y = [-1 0.154 0.528 0.912 0.887 1 0.873 0.955 0.592 0.147 -1];
drag_mach_x = [0 0.5 0.55 0.6 0.65 0.7 0.75 0.8 0.85 0.9 0.95 1 1.1 1.5]; drag_mach_y = [0 0 0 0 0 0 0 0 0 0 0.1 1 0.532 0.046];
CLde = -1.80648;
CD0 = 0.018;
CM0 = -0.06566;
CMde = -7.30733;
CMtrim = -7.30733;
trim_eff = 3;
AR = 8.461692097;
oswald = 0.75;
CL_drag_zero = 0.2;
alpha_deg = alpha_rad * 57.29577951308232;
CL_base = lookup1(lift_x, lift_y, alpha_rad);
CL = CL_base + CLde * elevator_rad;
CD_mach = lookup1(drag_mach_x, drag_mach_y, mach);
CD_induced = (CL - CL_drag_zero) * (CL - CL_drag_zero) / (3.141592653589793 * AR * oswald);
CD = CD0 + CD_induced + CD_mach;
elev_eff = lookup1(elev_eff_x, elev_eff_y, alpha_deg);
CM_alpha = CM0 + lookup1(pitch_x, pitch_y, alpha_rad);
CM = CM_alpha + CMde * elevator_rad * elev_eff + CMtrim * elevator_trim_rad * trim_eff;
end

function v = lookup1(xbp, ybp, x)
x = min(max(x, xbp(1)), xbp(end));
idx = findInterval(xbp, x);
x1 = xbp(idx); x2 = xbp(idx+1);
t = 0.0;
if x2 ~= x1
    t = (x - x1) / (x2 - x1);
end
v = ybp(idx) + t * (ybp(idx+1) - ybp(idx));
end

function v = lookup2(xbp, ybp, table, x, y)
x = min(max(x, xbp(1)), xbp(end));
y = min(max(y, ybp(1)), ybp(end));
ix = findInterval(xbp, x);
iy = findInterval(ybp, y);
x1 = xbp(ix); x2 = xbp(ix+1);
y1 = ybp(iy); y2 = ybp(iy+1);
tx = 0.0; ty = 0.0;
if x2 ~= x1
    tx = (x - x1) / (x2 - x1);
end
if y2 ~= y1
    ty = (y - y1) / (y2 - y1);
end
q11 = table(ix, iy);
q21 = table(ix+1, iy);
q12 = table(ix, iy+1);
q22 = table(ix+1, iy+1);
v = (1-tx)*(1-ty)*q11 + tx*(1-ty)*q21 + (1-tx)*ty*q12 + tx*ty*q22;
end

function idx = findInterval(bp, x)
idx = 1;
for n = 1:(numel(bp)-1)
    if x >= bp(n) && x <= bp(n+1)
        idx = n;
        return;
    end
end
idx = numel(bp)-1;
end

== matlab function simulink_flightgear_control_trim_wind_5/Plane/大气环境/气压高度+摄氏度偏差版本 ==
  data: T output; p output; rho output; Hp input; a output; delta_ISA input; delta output; theta output; sigma output
% File: isa_atmosphere_pressure_altitude_delta.m
%
% 输入:
%   Hp        气压高度 / pressure altitude (m) [0–84.852 km]
%   delta_ISA 温度偏差 (°C)，比如 -40 表示 ISA -40
%
% 输出:
%   T     实际温度 (K)，即 T_ISA(Hp) + delta_ISA
%   p     静压 (Pa)，由气压高度按 ISA 标准大气确定
%   rho   实际密度 (kg/m^3)，由 p 和 T 计算
%   a     实际声速 (m/s)，由 T 计算
%
% 可选输出:
%   delta 压力比 p/p0
%   theta 温度比 T/T0
%   sigma 密度比 rho/rho0

function [T, p, rho, a, delta, theta, sigma] = isa_atmosphere_pressure_altitude_delta(Hp, delta_ISA)

    % 常数
    g0 = 9.80665;        % m/s^2
    R  = 287.05287;      % J/(kg·K)
    gamma = 1.4;         % 空气比热比

    p0 = 101325;         % Pa
    T0 = 288.15;         % K
    rho0 = 1.225;        % kg/m^3

    % ISA 分层参数
    % 注意：这里 Hp 按标准大气的高度层处理
    h_base = [0, 11000, 20000, 32000, 47000, 51000, 71000, 84852]; % m
    L      = [-0.0065, 0.0, 0.0010, 0.0028, 0.0, -0.0028, -0.0020]; % K/m

    % 输入检查
    if any(Hp(:) < 0) || any(Hp(:) > 84852)
        error('Hp must be within [0, 84852] m.');
    end

    % 允许 delta_ISA 为标量或与 Hp 同尺寸
    if isscalar(delta_ISA)
        delta_ISA = delta_ISA .* ones(size(Hp));
    elseif ~isequal(size(delta_ISA), size(Hp))
        error('delta_ISA must be scalar or the same size as Hp.');
    end

    % 初始化
    T_ISA = zeros(size(Hp));
    p     = zeros(size(Hp));

    % 对每一个气压高度计算 ISA 温度和 ISA 压力
    for i = 1:numel(Hp)

        h = Hp(i);

        % 这里不能加 delta_ISA
        % 因为 pressure altitude 对应的压力必须由标准 ISA 反算
        T_curr = T0;
        p_curr = p0;

        for j = 1:length(L)

            h1 = h_base(j);
            h2 = h_base(j+1);

            if h <= h2

                if L(j) == 0
                    % 等温层
                    T_layer = T_curr;
                    p(i) = p_curr * exp(-g0 * (h - h1) / (R * T_layer));
                else
                    % 温度梯度层
                    T_layer = T_curr + L(j) * (h - h1);
                    p(i) = p_curr * (T_layer / T_curr)^(-g0 / (R * L(j)));
                end

                T_ISA(i) = T_layer;
                break;

            else

                % 穿越完整一层，更新到下一层基准
                if L(j) == 0
                    T_next = T_curr;
                    p_curr = p_curr * exp(-g0 * (h2 - h1) / (R * T_curr));
                else
                    T_next = T_curr + L(j) * (h2 - h1);
                    p_curr = p_curr * (T_next / T_curr)^(-g0 / (R * L(j)));
                end

                T_curr = T_next;
            end
        end
    end

    % 实际温度：在气压高度对应的 ISA 温度基础上加 ΔISA
    T = T_ISA + delta_ISA;

    if any(T(:) <= 0)
        error('Computed temperature is non-physical. T must be greater than 0 K.');
    end

    % 用实际温度计算密度和声速
    rho = p ./ (R .* T);
    a   = sqrt(gamma * R .* T);

    % 常用无量纲比值
    delta = p ./ p0;       % 压力比
    theta = T ./ T0;       % 温度比
    sigma = rho ./ rho0;   % 密度比
end

== matlab function simulink_flightgear_control_trim_wind_5/Plane/发动机/Subsystem/Static thrust1 ==
  data: mach input; total_thrust_lbf output; n1_cmd_pct input; single_engine_thrust_lbf output; thrust_factor output; n1_used_pct output
function [total_thrust_lbf, single_engine_thrust_lbf, thrust_factor, n1_used_pct] = core(mach, n1_cmd_pct)
%#codegen
n1_bp = [0 20 25 30 35 40 45 50 55 60 65 70 75 80 85 90 95 100 105 110];
mach_bp = [0 0.45 0.9];
tf_tbl = [0 0 0;0.053978 0.034816 0.080724;0.072647 0.042137 0.153968;0.092571 0.055766 0.352444;0.114397 0.087857 0.382598;0.133584 0.129235 0.401433;0.163657 0.179995 0.424077;0.201611 0.227881 0.453427;0.247145 0.284959 0.489514;0.306598 0.357671 0.526682;0.404374 0.458374 0.565243;0.472288 0.53715 0.610145;0.543975 0.608862 0.67375;0.628349 0.697486 0.766623;0.735036 0.796225 0.857414;0.837808 0.906299 0.97479;0.956614 1.020258 1.083902;1.090953 1.156054 1.221156;1.234866 1.296368 1.35787;1.325555 1.380287 1.43502];
static_thrust = 66500;
thrust_scalar = 1;
thrust_limit = 1;
n1_used_pct = min(max(n1_cmd_pct, n1_bp(1)), n1_bp(end));
thrust_factor = lookup2(n1_bp, mach_bp, tf_tbl, n1_used_pct, mach);
single_engine_thrust_lbf = static_thrust * thrust_factor * thrust_scalar * thrust_limit;
total_thrust_lbf = 4.0 * single_engine_thrust_lbf;
end

function v = lookup1(xbp, ybp, x)
x = min(max(x, xbp(1)), xbp(end));
idx = findInterval(xbp, x);
x1 = xbp(idx); x2 = xbp(idx+1);
t = 0.0;
if x2 ~= x1
    t = (x - x1) / (x2 - x1);
end
v = ybp(idx) + t * (ybp(idx+1) - ybp(idx));
end

function v = lookup2(xbp, ybp, table, x, y)
x = min(max(x, xbp(1)), xbp(end));
y = min(max(y, ybp(1)), ybp(end));
ix = findInterval(xbp, x);
iy = findInterval(ybp, y);
x1 = xbp(ix); x2 = xbp(ix+1);
y1 = ybp(iy); y2 = ybp(iy+1);
tx = 0.0; ty = 0.0;
if x2 ~= x1
    tx = (x - x1) / (x2 - x1);
end
if y2 ~= y1
    ty = (y - y1) / (y2 - y1);
end
q11 = table(ix, iy);
q21 = table(ix+1, iy);
q12 = table(ix, iy+1);
q22 = table(ix+1, iy+1);
v = (1-tx)*(1-ty)*q11 + tx*(1-ty)*q21 + (1-tx)*ty*q12 + tx*ty*q22;
end

function idx = findInterval(bp, x)
idx = 1;
for n = 1:(numel(bp)-1)
    if x >= bp(n) && x <= bp(n+1)
        idx = n;
        return;
    end
end
idx = numel(bp)-1;
end
